simulink model "Lab02_Group06_model"  (R2022b)
settings: Solver=ode1  StartTime=0.0  StopTime=10  FixedStep=0.002  RelTol=1e-3  EnableMultiTasking=on
undefined symbols (not defined in the file): DiscIntNeverNeededParam, HIL
libraries: quarc_library x4
settings Model: SimulationMode=external  ExtModeTrigDuration=100000  Creator=hamzah.nadeem  LastModifiedBy=hamzah.nadeem
settings SolverCC: PositivePriorityOrder=on
settings RTWCC: Description=QUARC Win64 Target Using Toolchain  SystemTargetFile=quarc_win64.tlc  Toolchain=QUARC win64 | nmake (64-bit Windows)  BuildConfiguration=Faster Runs
settings STFCustomTargetCC: TargetLangStandard=C99 (ISO)  ConcurrentExecutionCompliant=on  GRTInterface=on  UseToolchainInfoCompliant=on  SystemTargetFile=quarc_win64.tlc
settings GRTTargetCC: ParMdlRefBuildCompliant=off  CompOptLevelCompliant=off  CombineOutputUpdateFcns=off  MatFileLogging=off  CPPClassGenCompliant=off  GRTInterface=on  ExtMode=on  ExtModeMexFile=quarc_comm

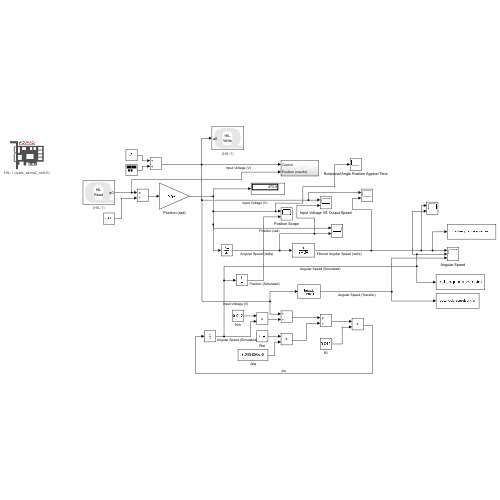
[thumbnail: Simulink's stored preview of the top-level diagram]
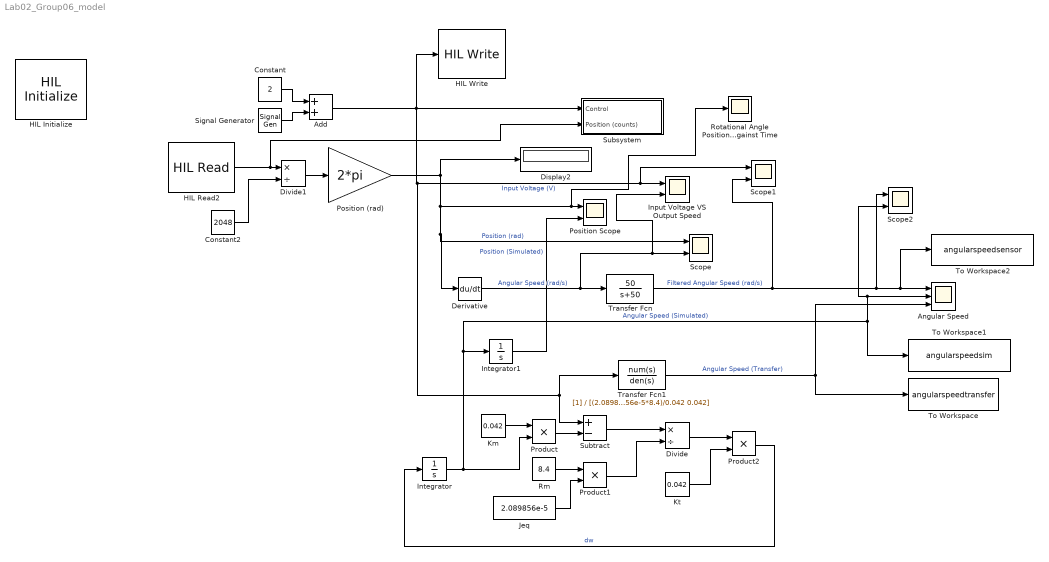
== system Lab02_Group06_model ==
  Add : Sum
  Angular Speed : Scope  NumInputPorts=3
  Constant : Constant  Value=2
  Constant2 : Constant  Value=2048
  Derivative : Derivative
  Display2 : Display
  Divide : Product  Inputs=*/  RndMeth=Zero  SaturateOnIntegerOverflow=on
  Divide1 : Product  Inputs=*/  RndMeth=Zero  SaturateOnIntegerOverflow=on
  HIL Initialize : quarc_library/Data Acquisition/Generic/Configuration/HIL Initialize  object_name=HIL-1  board_type=qube_servo2_usb  board_number=0  board_options=""  exclusive=off  active=on  hardware_clocks=[0]  clock_modes=[]  initial_clock_frequencies=[]  set_clock_params_at_start=off  set_clock_params_at_switch_in=off  set_clock_frequencies_at_start=off  set_clock_frequencies_at_switch_in=off  analog_input_channels=[0]  analog_input_configurations=[]  analog_input_maximums=3  analog_input_minimums=-3  set_analog_input_params_at_start=off  set_analog_input_params_at_switch_in=off  analog_output_channels=[0]  analog_output_maximums=15  analog_output_minimums=-15  initial_analog_outputs=[0]  final_analog_outputs=[0]  watchdog_analog_outputs=0  set_analog_output_params_at_start=off  set_analog_output_params_at_switch_in=off  set_analog_outputs_at_start=on  set_analog_outputs_at_switch_in=off  set_analog_outputs_at_terminate=on  set_analog_outputs_at_switch_out=off  set_analog_outputs_on_watchdog=on  digital_input_channels=[]  digital_output_channels=[0]  digital_output_configuration=[]  initial_digital_outputs=[1]  final_digital_outputs=[0]  watchdog_digital_outputs=[0]  set_digital_output_params_at_start=off  set_digital_output_params_at_switch_in=off  set_digital_outputs_at_start=on  set_digital_outputs_at_switch_in=off  set_digital_outputs_at_terminate=on  set_digital_outputs_at_switch_out=off  set_digital_outputs_on_watchdog=on  encoder_channels=[0:1]  quadrature=[4]  encoder_filter_frequency=[]  initial_encoder_counts=[0]  set_encoder_params_at_start=off  set_encoder_params_at_switch_in=off  set_encoder_counts_at_start=on  set_encoder_counts_at_switch_in=off  pwm_channels=[]  pwm_modes=[]  pwm_frequency=[]  pwm_configuration=[]  pwm_alignment=[]  pwm_polarity=[]  pwm_leading_deadband=[]  pwm_trailing_deadband=[]  initial_pwm_outputs=[]  final_pwm_outputs=[]  watchdog_pwm_outputs=[]  set_pwm_params_at_start=off  set_pwm_params_at_switch_in=off  set_pwm_outputs_at_start=off  set_pwm_outputs_at_switch_in=off  set_pwm_outputs_at_terminate=off  set_pwm_outputs_at_switch_out=off  set_pwm_outputs_on_watchdog=off  other_output_channels=[11000:11002]  initial_other_outputs=[0 1 0]  final_other_outputs=[1 0 0]  watchdog_other_outputs=[0 0 1]  set_other_outputs_at_start=on  set_other_outputs_at_switch_in=off  set_other_outputs_at_terminate=on  set_other_outputs_at_switch_out=off  set_other_outputs_on_watchdog=on
  HIL Read2 : quarc_library/Data Acquisition/Generic/Immediate I//O/HIL Read  object_name=HIL-1  analog_channels=[]  encoder_channels=0  digital_channels=[]  other_channels=[]  sample_time=qc_get_step_size  active=on  vector_output=off  data_type_mode=Inherit via back propagation  encoder_data_type=double  digital_data_type=boolean
  HIL Write : quarc_library/Data Acquisition/Generic/Immediate I//O/HIL Write  object_name=HIL-1  analog_channels=0  pwm_channels=[]  digital_channels=[]  other_channels=[]  sample_time=-1  active=off  vector_input=off
  Input Voltage VS Output Speed : Scope  NumInputPorts=2
  Integrator : Integrator
  Integrator1 : Integrator
  Jeq : Constant  Value=2.089856e-5
  Km : Constant  Value=0.042
  Kt : Constant  Value=0.042
  Position (rad) : Gain  Gain=2*pi
  Position Scope : Scope  NumInputPorts=2
  Product : Product
  Product1 : Product
  Product2 : Product
  Rm : Constant  Value=8.4
  Rotational Angle Position Against Time : Scope
  Scope : Scope  NumInputPorts=2
  Scope1 : Scope  NumInputPorts=2
  Scope2 : Scope  NumInputPorts=2
  Signal Generator : SignalGenerator  WaveForm=square  Frequency=0.4
  Subsystem : Subsystem
  Subtract : Sum  Inputs=+-
  To Workspace : ToWorkspace  VariableName=angularspeedtransfer  SampleTime=-1
  To Workspace1 : ToWorkspace  VariableName=angularspeedsim  SampleTime=-1
  To Workspace2 : ToWorkspace  VariableName=angularspeedsensor  SampleTime=-1
  Transfer Fcn : TransferFcn  Numerator=[50]  Denominator=[1 50]
  Transfer Fcn1 : TransferFcn  Denominator=[(2.089856e-5*8.4)/0.042 0.042]
  wires:
  Divide1/1 -> Position (rad)/1
  HIL Read2/1 -> Subsystem/2(Position (counts)), Divide1/1
  Constant2/1 -> Divide1/2
  Position (rad)/1 -> Derivative/1, Scope/1, Rotational Angle Position Against Time/1, Position Scope/1, Display2/1  "Position (rad)"
  Add/1 -> Subtract/1, Transfer Fcn1/1, Scope1/1, Input Voltage VS Output Speed/1, Subsystem/1(Control), HIL Write/1  "Input Voltage (V)"
  Derivative/1 -> Transfer Fcn/1, Input Voltage VS Output Speed/2, Scope/2  "Angular Speed (rad/s)"
  Product/1 -> Subtract/2
  Product1/1 -> Divide/2
  Jeq/1 -> Product1/2
  Rm/1 -> Product1/1
  Km/1 -> Product/1
  Subtract/1 -> Divide/1
  Kt/1 -> Product2/2
  Divide/1 -> Product2/1
  Integrator/1 -> To Workspace1/1, Angular Speed/2, Scope2/2, Integrator1/1, Product/2  "Angular Speed (Simulated)"
  Product2/1 -> Integrator/1  "dw"
  Integrator1/1 -> Position Scope/2  "Position (Simulated)"
  Constant/1 -> Add/1
  Signal Generator/1 -> Add/2
  Transfer Fcn1/1 -> Angular Speed/3, To Workspace/1  "Angular Speed (Transfer)"
  Transfer Fcn/1 -> Scope1/2, Scope2/1, To Workspace2/1, Angular Speed/1  "Filtered Angular Speed (rad/s)"

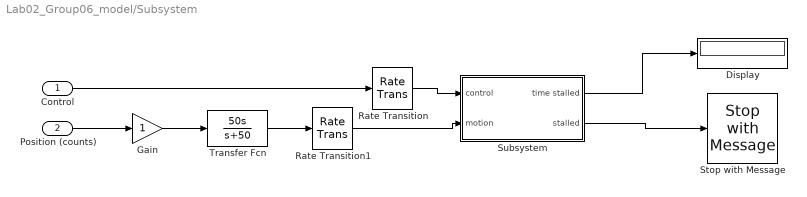
== system Lab02_Group06_model/Subsystem ==
  Control : Inport
  Position (counts) : Inport  Port=2
  Display : Display
  Gain : Gain
  Rate Transition : RateTransition
  Rate Transition1 : RateTransition
  Stop with Message : quarc_library/Sinks/Error Handling/Stop with Message  message_type=Fixed error message  message_icon=Error  message=Stall Detected! Please snsure that the DC motor is free to move and is functioning properly. Please ask a TA to check your code if you have recived this error.
  Subsystem : Subsystem
  Transfer Fcn : TransferFcn  Numerator=[50 0]  Denominator=[1 50]
  wires:
  Subsystem/2(stalled) -> Stop with Message/1
  Subsystem/1(time stalled) -> Display/1
  Rate Transition/1 -> Subsystem/1(control)
  Rate Transition1/1 -> Subsystem/2(motion)
  Transfer Fcn/1 -> Rate Transition1/1
  Gain/1 -> Transfer Fcn/1
  Position (counts)/1 -> Gain/1
  Control/1 -> Rate Transition/1

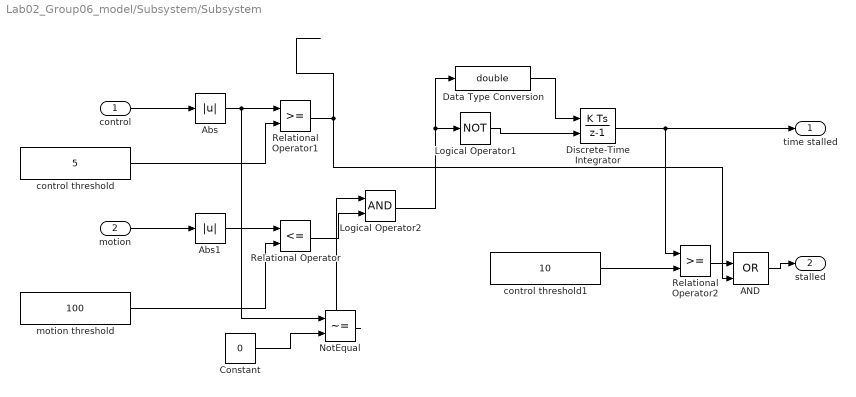
== system Lab02_Group06_model/Subsystem/Subsystem ==
  control : Inport
  motion : Inport  Port=2
  AND : Logic  Operator=OR  IconShape=distinctive  AllPortsSameDT=off  OutDataTypeStr=boolean
  Abs : Abs  SaturateOnIntegerOverflow=off
  Abs1 : Abs  SaturateOnIntegerOverflow=off
  Constant : Constant  Value=0
  Data Type Conversion : DataTypeConversion  OutDataTypeStr=double  SaturateOnIntegerOverflow=off  RndMeth=Floor
  Discrete-Time Integrator : DiscreteIntegrator  ExternalReset=rising  SampleTime=-1  ICPrevOutput=DiscIntNeverNeededParam  ICPrevScaledInput=DiscIntNeverNeededParam
  Logical Operator1 : Logic  Operator=NOT  AllPortsSameDT=off  OutDataTypeStr=boolean
  Logical Operator2 : Logic  AllPortsSameDT=off  OutDataTypeStr=boolean
  NotEqual : RelationalOperator  Operator=~=  OutDataTypeStr=boolean  RndMeth=Simplest  InputSameDT=off
  Relational Operator : RelationalOperator  Operator=<=  OutDataTypeStr=boolean  InputSameDT=off
  Relational Operator1 : RelationalOperator  OutDataTypeStr=boolean  InputSameDT=off
  Relational Operator2 : RelationalOperator  OutDataTypeStr=boolean  InputSameDT=off
  control threshold : Constant  Value=5
  control threshold1 : Constant  Value=10
  motion threshold : Constant  Value=100
  time stalled : Outport
  stalled : Outport  Port=2
  wires:
  NotEqual/1 -> Logical Operator2/1
  Relational Operator/1 -> Logical Operator2/2
  AND/1 -> stalled/1
  Relational Operator2/1 -> AND/1
  Relational Operator1/1 -> AND/2
  Constant/1 -> NotEqual/2
  control threshold1/1 -> Relational Operator2/2
  Abs1/1 -> Relational Operator/1
  Data Type Conversion/1 -> Discrete-Time Integrator/1
  Discrete-Time Integrator/1 -> Relational Operator2/1, time stalled/1
  Logical Operator1/1 -> Discrete-Time Integrator/2
  control/1 -> Abs/1
  Abs/1 -> Relational Operator1/1, NotEqual/1
  control threshold/1 -> Relational Operator1/2
  motion threshold/1 -> Relational Operator/2
  Logical Operator2/1 -> Data Type Conversion/1, Logical Operator1/1
  motion/1 -> Abs1/1
